simulink model "CSTR_Simulink"  (R2026a)
settings: Solver=ode15s  StopTime=model.time  FixedStep=5./60./10000
values from neighbouring files (symbols this model uses):
  A = 16.66    [plant_data_gen.m]
  Cv_Q = SS.Q ./ ( SS.lQ .* N .* sqrt( ( SS.P_U - SS.P_D ) ./ g_s) )    [plant_data_gen.m]
  Cv_Q_C = SS.Q_C ./ ( SS.lQ_C .* N .* sqrt( ( SS.P_CU - SS.P_CD ) ./ g_s ) )    [plant_data_gen.m]
  deltaH = -5e4    (= -50000)    [plant_data_gen.m]
  EoR = 8750    [plant_data_gen.m]
  g_s = 1    [plant_data_gen.m]
  K = size(x)    [PPCA_validation.m]    (also in plant_data_gen.m = 0.0625)
  k_0 = 7.2e10    (= 72000000000)    [plant_data_gen.m]
  Kc_h = -3.0    (= -3)    [plant_data_gen.m]
  Kc_Q = 0.2    [plant_data_gen.m]
  Kc_Q_C = 0.2    [plant_data_gen.m]
  Kc_T = -2.0    (= -2)    [plant_data_gen.m]
  Km_Q = 8/100    (= 0.08)    [plant_data_gen.m]
  Km_Q_C = 8/15    (= 0.533333333333)    [plant_data_gen.m]
  N = 0.0865 * 1000 / 60 / sqrt(1000)    [plant_data_gen.m]
  rhoCp = 239    [plant_data_gen.m]
  rhoCp_C = 4175    [plant_data_gen.m]
  tau = 2./60    (= 0.0333333333333)    [plant_data_gen.m]
  TI_h = 1./TI_h    (= 0.666666666667)    [plant_data_gen.m]
  TI_Q = 1.7/60    (= 0.0283333333333)    [plant_data_gen.m]
  TI_Q_C = 1./TI_Q_C    (= 35.2941176471)    [plant_data_gen.m]
  TI_T = 1./TI_T    (= 1.14942528736)    [plant_data_gen.m]
  UA_C = 5e4    (= 50000)    [plant_data_gen.m]
  V_C = 10    [plant_data_gen.m]
undefined symbols (not defined in the file or in its folder): D, model, noise, SS
libraries: dspsrcs4 x16, simulink x8, slpidlib x4
(part 2 of 2)

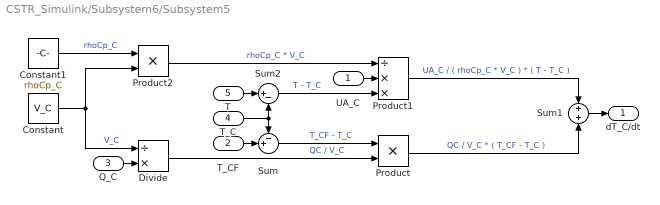
== system CSTR_Simulink/Subsystem6/Subsystem5 ==
  UA_C : Inport
  T_CF : Inport  Port=2
  Q_C : Inport  Port=3
  T_C : Inport  Port=4
  T : Inport  Port=5
  Constant : Constant  Value=V_C
  Constant1 : Constant  Value=rhoCp_C
  Divide : Product  Inputs=/*
  Product : Product
  Product1 : Product  Inputs=/**
  Product2 : Product
  Sum : Sum  Inputs=-+|
  Sum1 : Sum  Inputs=+|+
  Sum2 : Sum  Inputs=|+-
  dT_C/dt : Outport
  wires:
  Divide/1 -> Product/2  "QC / V_C"
  Constant/1 -> Divide/1, Product2/2  "V_C"
  Product1/1 -> Sum1/1  "UA_C / ( rhoCp_C * V_C ) * ( T - T_C )"
  Constant1/1 -> Product2/1  "rhoCp_C"
  Product2/1 -> Product1/1  "rhoCp_C * V_C"
  Product/1 -> Sum1/2  "QC / V_C * ( T_CF - T_C )"
  T_C/1 -> Sum/1, Sum2/2
  Sum/1 -> Product/1  "T_CF - T_C"
  UA_C/1 -> Product1/2
  T/1 -> Sum2/1
  T_CF/1 -> Sum/2
  Q_C/1 -> Divide/2
  Sum1/1 -> dT_C/dt/1
  Sum2/1 -> Product1/3  "T - T_C"
